simulink model "trackingLinSim"  (R2021b)
settings: Solver=VariableStepAuto  StartTime=0.0  StopTime=100  RelTol=1e-3
values from neighbouring files (symbols this model uses):
  A = [-0.0665 -11.4608 0.1439 -32.1740 ... (first row only)    [Dorobantu.m]    (also in exampleRSS.m = rss(1,1,1); lpvExample.m = [0.75 2 cos(rhoData(i)) sin(rhoData(i));0 0.5 -sin(rhoData(i)
  B = [0.1419 -0.0435 ... (first row only)    [Dorobantu.m]    (also in lpvExample.m = [0 0 0;a 0 0;0 10 0;0 0 10])
  C = eye(4)    [Dorobantu.m]    (also in lpvExample.m = [1 0 0 0;0 1 0 0])
  D = zeros(4,2)    [Dorobantu.m]    (also in lpvExample.m = zeros(2,3))
  g = 32.17405    [SingleDOF.m]    (also in layer1atm.m; mainSimple.m = 32.174; simio.m = [dx(Index.EOM(1:6)); delta(:)-f; -delta(:)-f ])
  K_lon_hinf = pss(K_lon_hinfs,Domain)    [SingleDOF.m]    (also in main.m; mainSimple.m)
  LTI_lon = ss(A,B,C,D)    [Dorobantu.m]    (also in mainLinear.m = GTM_lon(:,:,i,j,k); newmain.m = GTM_lon(:,:,i,j,k))
  s = tf('s')    [SingleDOF.m]    (also in main.m; mainSimple.m; newmain.m)
undefined symbols (not defined in the file or in its folder): ft
libraries: simulink_extras x4, aerolibconvert2 x2
settings Model: Creator=jihoo  LastModifiedBy=jihoo

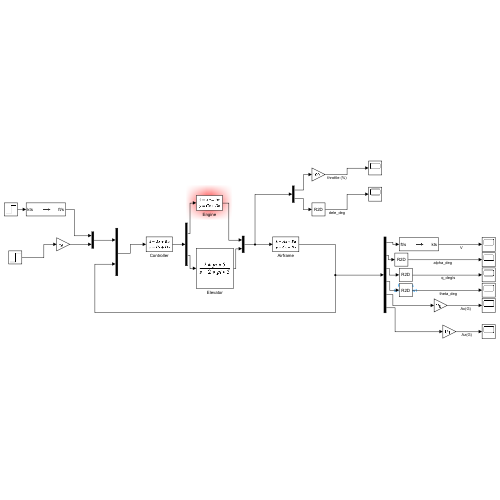
[thumbnail: Simulink's stored preview of the top-level diagram]
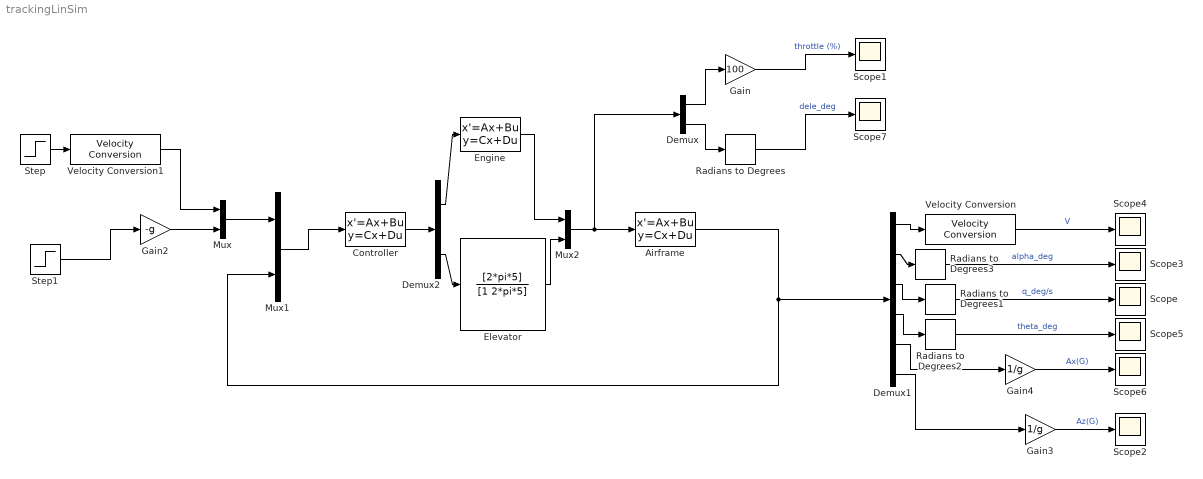
== system trackingLinSim ==
  Airframe : StateSpace  A=LTI_lon.A  B=LTI_lon.B  C=LTI_lon.C  D=LTI_lon.D  InitialCondition=0
  Controller : StateSpace  A=K_lon_hinf.A  B=K_lon_hinf.B  C=K_lon_hinf.C  D=K_lon_hinf.D  InitialCondition=0
  Demux : Demux  Outputs=2
  Demux1 : Demux  Outputs=6
  Demux2 : Demux  Outputs=2
  Elevator : TransferFcn  Numerator=[2*pi*5]  Denominator=[1 2*pi*5]
  Engine : StateSpace  A=A  B=B  C=C  D=D  InitialCondition=0
  Gain : Gain  Gain=100
  Gain2 : Gain  Gain=-g
  Gain3 : Gain  Gain=1/g
  Gain4 : Gain  Gain=1/g
  Mux : Mux  Inputs=2
  Mux1 : Mux  Inputs=2
  Mux2 : Mux  Inputs=2
  Radians to Degrees{,1..3} (4 alike) : simulink_extras/Transformations/Radians to Degrees
  Scope{,1..7} (8 alike) : Scope
  Step : Step  Time=0  After=0  SampleTime=0
  Step1 : Step  SampleTime=0
  Velocity Conversion : aerolibconvert2/Velocity Conversion  IU=ft/s  OU=kts
  Velocity Conversion1 : aerolibconvert2/Velocity Conversion  IU=kts  OU=ft/s
  wires:
  Velocity Conversion1/1 -> Mux/1
  Gain2/1 -> Mux/2
  Gain/1 -> Scope1/1  "throttle (%)"
  Demux1/1 -> Velocity Conversion/1
  Radians to Degrees1/1 -> Scope/1  "q_deg/s"
  Radians to Degrees/1 -> Scope7/1  "dele_deg"
  Airframe/1 -> Demux1/1, Mux1/2
  Demux/2 -> Radians to Degrees/1
  Radians to Degrees2/1 -> Scope5/1  "theta_deg"
  Mux2/1 -> Demux/1, Airframe/1
  Demux/1 -> Gain/1
  Velocity Conversion/1 -> Scope4/1  "V"
  Mux/1 -> Mux1/1
  Radians to Degrees3/1 -> Scope3/1  "alpha_deg"
  Demux1/5 -> Gain4/1
  Mux1/1 -> Controller/1
  Step/1 -> Velocity Conversion1/1
  Step1/1 -> Gain2/1
  Demux1/4 -> Radians to Degrees2/1
  Demux1/3 -> Radians to Degrees1/1
  Demux1/2 -> Radians to Degrees3/1
  Demux1/6 -> Gain3/1
  Gain3/1 -> Scope2/1  "Az(G)"
  Gain4/1 -> Scope6/1  "Ax(G)"
  Controller/1 -> Demux2/1
  Demux2/1 -> Engine/1
  Engine/1 -> Mux2/1
  Demux2/2 -> Elevator/1
  Elevator/1 -> Mux2/2
